simulink model "N4Diag"  (R2024b)
settings: Solver=ode45  StartTime=0.0  StopTime=2  RelTol=1e-3
values from neighbouring files (symbols this model uses):
  T = 10e-3    (= 0.01)    [AnalisisReg.m]    (also in regdiagsep.m = Reg.Ts)
undefined symbols (not defined in the file or in its folder): DiscIntNeverNeededParam, N, RegDiagA_Len2_ext, RegDiagA_Len3_ext, RegDiagA_Len4_ext, RegDiagB_Len2_ext, RegDiagB_Len3_ext, RegDiagB_Len4_ext, RegDiagC_Len2_ext, RegDiagC_Len3_ext, RegDiagC_Len4_ext, RegDiagD_Len2_ext, RegDiagD_Len3_ext, RegDiagD_Len4_ext, RegDiagE_Len2_ext, RegDiagE_Len3_ext, RegDiagE_Len4_ext, RegDiagF_Len2_ext, RegDiagF_Len3_ext, RegDiagF_Len4_ext, RegDiagG_Len2_ext, RegDiagG_Len3_ext, RegDiagG_Len4_ext
libraries: cstblocks x27
settings Model: Creator=Guillem  LastModifiedBy=jroigro
settings SolverCC: AlgebraicLoopSolver=TrustRegion
settings DataIOCC: LimitDataPoints=on  SaveFormat=Array  SignalLoggingSaveFormat=ModelDataLogs  ReturnWorkspaceOutputs=off
settings OptimizationCC: BlockReduction=off  BooleanDataType=off  LifeSpan=inf
settings DebuggingCC: SaveWithParameterizedLinksMsg=none  UnderspecifiedInitializationDetection=Classic  MergeDetectMultiDrivingBlocksExec=none  SignalResolutionControl=TryResolveAllWithWarning  MultiTaskDSMMsg=warning  MultiTaskCondExecSysMsg=none  UnconnectedInputMsg=warning  UnconnectedOutputMsg=warning  UnconnectedLineMsg=warning  SFUnexpectedBacktrackingDiag=warning  SFNoUnconditionalDefaultTransitionDiag=warning  SFExecutionAtInitializationDiag=none  ArithmeticOperatorsInVariantConditions=warning
settings HardwareCC: ProdBitPerPointer=32  ProdBitPerSizeT=32  ProdBitPerPtrDiffT=32  ProdLargestAtomicFloat=None  ProdIntDivRoundTo=Undefined  ProdEndianess=Unspecified  ProdWordSize=32  ProdHWDeviceType=32-bit Generic  TargetUnknown=on
settings ModelReferenceCC: PropagateSignalLabelsOutOfModel=off
settings SFSimCC: SimUseLocalCustomCode=off  CustomCodeUndefinedFunction=UseInterfaceOnly
settings RTWCC: RTWUseLocalCustomCode=off  GPUComputeCapability=3.5
settings CodeAppCC: StateflowObjectComments=on
settings GRTTargetCC: TargetLangStandard=C89/C90 (ANSI)
settings ConfigComp: CovMetricSettings=dw  CovSaveCumulativeToWorkspaceVar=on  CovSaveSingleToWorkspaceVar=on  CovExternalEMLEnable=off

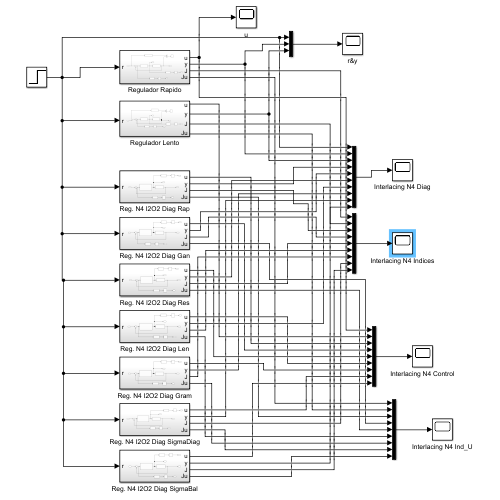
[thumbnail: Simulink's stored preview of the top-level diagram]
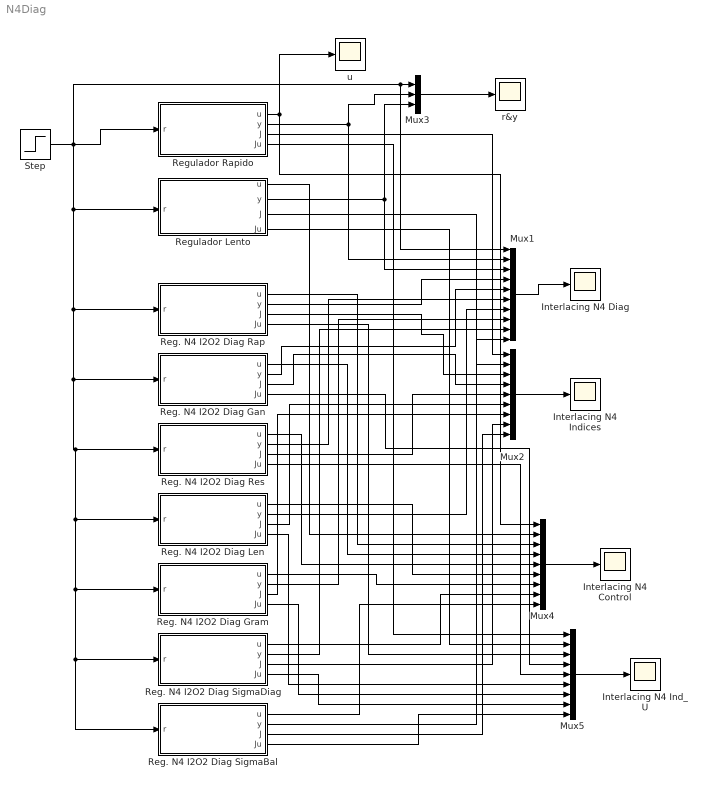
== system N4Diag ==
  Interlacing N4 Control : Scope
  Interlacing N4 Diag : Scope
  Interlacing N4 Ind_U : Scope
  Interlacing N4 Indices : Scope
  Mux1 : Mux  Inputs=10
  Mux2 : Mux  Inputs=9
  Mux3 : Mux  Inputs=3
  Mux4 : Mux  Inputs=9
  Mux5 : Mux  Inputs=9
  Reg. N4 I2O2 Diag Gan : Subsystem
  Reg. N4 I2O2 Diag Gram : Subsystem
  Reg. N4 I2O2 Diag Len : Subsystem
  Reg. N4 I2O2 Diag Rap : Subsystem
  Reg. N4 I2O2 Diag Res : Subsystem
  Reg. N4 I2O2 Diag SigmaBal : Subsystem
  Reg. N4 I2O2 Diag SigmaDiag : Subsystem
  Regulador Lento : Subsystem
  Regulador Rapido : Subsystem
  Step : Step  Time=10  Before=1  After=2  SampleTime=0
  r&y : Scope
  u : Scope
  wires:
  Mux3/1 -> r&y/1
  Regulador Rapido/2(y) -> Mux1/2, Mux3/2
  Regulador Rapido/1(u) -> Mux4/1, u/1
  Mux1/1 -> Interlacing N4 Diag/1
  Regulador Lento/2(y) -> Mux1/3, Mux3/3
  Reg. N4 I2O2 Diag Rap/2(y) -> Mux1/4
  Reg. N4 I2O2 Diag Gan/2(y) -> Mux1/5
  Reg. N4 I2O2 Diag Res/2(y) -> Mux1/6
  Reg. N4 I2O2 Diag Len/2(y) -> Mux1/7
  Mux2/1 -> Interlacing N4 Indices/1
  Regulador Rapido/3(J) -> Mux2/1
  Regulador Lento/3(J) -> Mux2/2
  Reg. N4 I2O2 Diag Rap/3(J) -> Mux2/3
  Reg. N4 I2O2 Diag Gan/3(J) -> Mux2/4
  Reg. N4 I2O2 Diag Res/3(J) -> Mux2/5
  Reg. N4 I2O2 Diag Len/3(J) -> Mux2/6
  Reg. N4 I2O2 Diag Gram/3(J) -> Mux2/7
  Step/1 -> Reg. N4 I2O2 Diag SigmaBal/1(r), Reg. N4 I2O2 Diag SigmaDiag/1(r), Reg. N4 I2O2 Diag Gram/1(r), Reg. N4 I2O2 Diag Len/1(r), Reg. N4 I2O2 Diag Res/1(r), Reg. N4 I2O2 Diag Gan/1(r), Reg. N4 I2O2 Diag Rap/1(r), Regulador Lento/1(r), Mux1/1, Mux3/1, Regulador Rapido/1(r)
  Reg. N4 I2O2 Diag Gram/2(y) -> Mux1/8
  Mux4/1 -> Interlacing N4 Control/1
  Regulador Lento/1(u) -> Mux4/2
  Reg. N4 I2O2 Diag Rap/1(u) -> Mux4/3
  Reg. N4 I2O2 Diag Gan/1(u) -> Mux4/4
  Reg. N4 I2O2 Diag Res/1(u) -> Mux4/5
  Reg. N4 I2O2 Diag Len/1(u) -> Mux4/6
  Reg. N4 I2O2 Diag Gram/1(u) -> Mux4/7
  Reg. N4 I2O2 Diag SigmaDiag/1(u) -> Mux4/8
  Reg. N4 I2O2 Diag SigmaBal/1(u) -> Mux4/9
  Reg. N4 I2O2 Diag SigmaDiag/2(y) -> Mux1/9
  Reg. N4 I2O2 Diag SigmaBal/2(y) -> Mux1/10
  Reg. N4 I2O2 Diag SigmaDiag/3(J) -> Mux2/8
  Reg. N4 I2O2 Diag SigmaBal/3(J) -> Mux2/9
  Mux5/1 -> Interlacing N4 Ind_U/1
  Reg. N4 I2O2 Diag SigmaBal/4(Ju) -> Mux5/9
  Reg. N4 I2O2 Diag SigmaDiag/4(Ju) -> Mux5/8
  Reg. N4 I2O2 Diag Gram/4(Ju) -> Mux5/7
  Reg. N4 I2O2 Diag Len/4(Ju) -> Mux5/6
  Reg. N4 I2O2 Diag Res/4(Ju) -> Mux5/5
  Reg. N4 I2O2 Diag Gan/4(Ju) -> Mux5/4
  Reg. N4 I2O2 Diag Rap/4(Ju) -> Mux5/3
  Regulador Lento/4(Ju) -> Mux5/2
  Regulador Rapido/4(Ju) -> Mux5/1

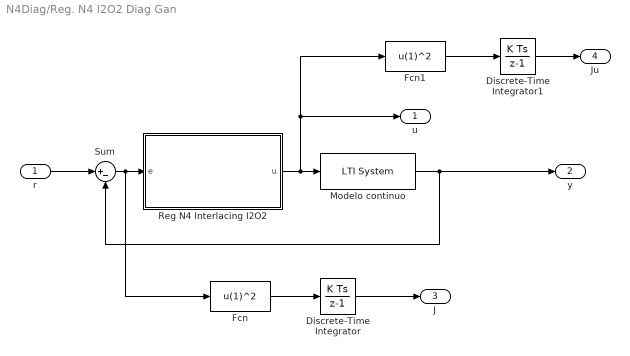
== system N4Diag/Reg. N4 I2O2 Diag Gan ==
  r : Inport
  Discrete-Time Integrator : DiscreteIntegrator  gainval=1/T  SampleTime=T  ICPrevOutput=DiscIntNeverNeededParam  ICPrevScaledInput=DiscIntNeverNeededParam
  Discrete-Time Integrator1 : DiscreteIntegrator  gainval=1/T  SampleTime=T  ICPrevOutput=DiscIntNeverNeededParam  ICPrevScaledInput=DiscIntNeverNeededParam
  Fcn : Fcn  Expr=u(1)^2
  Fcn1 : Fcn  Expr=u(1)^2
  Modelo continuo : cstblocks/LTI System  sys=Planta  IC=[]  PadeOrder=0
  Reg N4 Interlacing I2O2 : Subsystem
  Sum : Sum  Inputs=|+-
  u : Outport
  y : Outport  Port=2
  J : Outport  Port=3
  Ju : Outport  Port=4
  wires:
  r/1 -> Sum/1
  Reg N4 Interlacing I2O2/1(u) -> Fcn1/1, u/1, Modelo continuo/1
  Modelo continuo/1 -> y/1, Sum/2
  Sum/1 -> Fcn/1, Reg N4 Interlacing I2O2/1(e)
  Fcn/1 -> Discrete-Time Integrator/1
  Discrete-Time Integrator/1 -> J/1
  Fcn1/1 -> Discrete-Time Integrator1/1
  Discrete-Time Integrator1/1 -> Ju/1

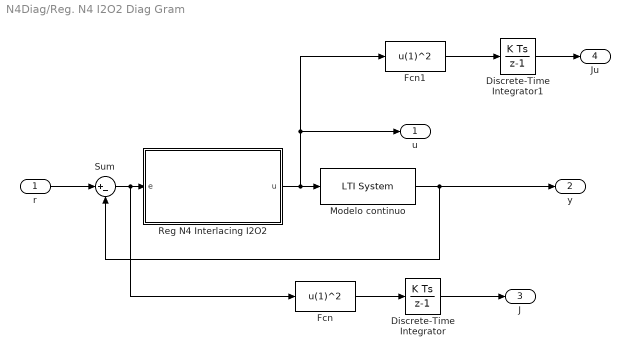
== system N4Diag/Reg. N4 I2O2 Diag Gram ==
  r : Inport
  Discrete-Time Integrator : DiscreteIntegrator  gainval=1/T  SampleTime=T  ICPrevOutput=DiscIntNeverNeededParam  ICPrevScaledInput=DiscIntNeverNeededParam
  Discrete-Time Integrator1 : DiscreteIntegrator  gainval=1/T  SampleTime=T  ICPrevOutput=DiscIntNeverNeededParam  ICPrevScaledInput=DiscIntNeverNeededParam
  Fcn : Fcn  Expr=u(1)^2
  Fcn1 : Fcn  Expr=u(1)^2
  Modelo continuo : cstblocks/LTI System  sys=Planta  IC=[]  PadeOrder=0
  Reg N4 Interlacing I2O2 : Subsystem
  Sum : Sum  Inputs=|+-
  u : Outport
  y : Outport  Port=2
  J : Outport  Port=3
  Ju : Outport  Port=4
  wires:
  Discrete-Time Integrator/1 -> J/1
  Fcn/1 -> Discrete-Time Integrator/1
  Sum/1 -> Reg N4 Interlacing I2O2/1(e), Fcn/1
  Modelo continuo/1 -> Sum/2, y/1
  r/1 -> Sum/1
  Fcn1/1 -> Discrete-Time Integrator1/1
  Reg N4 Interlacing I2O2/1(u) -> Modelo continuo/1, Fcn1/1, u/1
  Discrete-Time Integrator1/1 -> Ju/1

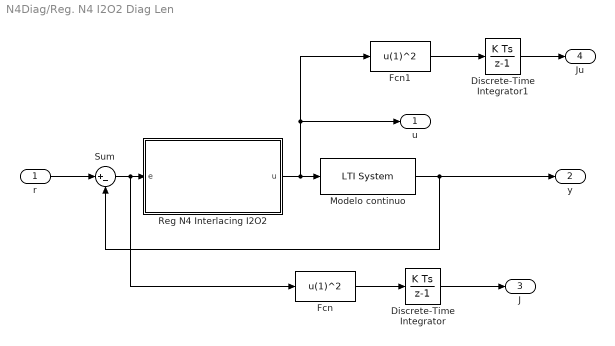
== system N4Diag/Reg. N4 I2O2 Diag Len ==
  r : Inport
  Discrete-Time Integrator : DiscreteIntegrator  gainval=1/T  SampleTime=T  ICPrevOutput=DiscIntNeverNeededParam  ICPrevScaledInput=DiscIntNeverNeededParam
  Discrete-Time Integrator1 : DiscreteIntegrator  gainval=1/T  SampleTime=T  ICPrevOutput=DiscIntNeverNeededParam  ICPrevScaledInput=DiscIntNeverNeededParam
  Fcn : Fcn  Expr=u(1)^2
  Fcn1 : Fcn  Expr=u(1)^2
  Modelo continuo : cstblocks/LTI System  sys=Planta  IC=[]  PadeOrder=0
  Reg N4 Interlacing I2O2 : Subsystem
  Sum : Sum  Inputs=|+-
  u : Outport
  y : Outport  Port=2
  J : Outport  Port=3
  Ju : Outport  Port=4
  wires:
  r/1 -> Sum/1
  Modelo continuo/1 -> y/1, Sum/2
  Sum/1 -> Fcn/1, Reg N4 Interlacing I2O2/1(e)
  Fcn/1 -> Discrete-Time Integrator/1
  Discrete-Time Integrator/1 -> J/1
  Fcn1/1 -> Discrete-Time Integrator1/1
  Reg N4 Interlacing I2O2/1(u) -> Fcn1/1, u/1, Modelo continuo/1
  Discrete-Time Integrator1/1 -> Ju/1

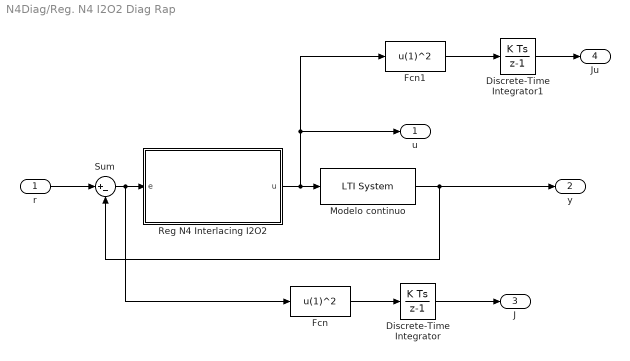
== system N4Diag/Reg. N4 I2O2 Diag Rap ==
  r : Inport
  Discrete-Time Integrator : DiscreteIntegrator  gainval=1/T  SampleTime=T  ICPrevOutput=DiscIntNeverNeededParam  ICPrevScaledInput=DiscIntNeverNeededParam
  Discrete-Time Integrator1 : DiscreteIntegrator  gainval=1/T  SampleTime=T  ICPrevOutput=DiscIntNeverNeededParam  ICPrevScaledInput=DiscIntNeverNeededParam
  Fcn : Fcn  Expr=u(1)^2
  Fcn1 : Fcn  Expr=u(1)^2
  Modelo continuo : cstblocks/LTI System  sys=Planta  IC=[]  PadeOrder=0
  Reg N4 Interlacing I2O2 : Subsystem
  Sum : Sum  Inputs=|+-
  u : Outport
  y : Outport  Port=2
  J : Outport  Port=3
  Ju : Outport  Port=4
  wires:
  Modelo continuo/1 -> Sum/2, y/1
  r/1 -> Sum/1
  Sum/1 -> Fcn/1, Reg N4 Interlacing I2O2/1(e)
  Fcn/1 -> Discrete-Time Integrator/1
  Discrete-Time Integrator/1 -> J/1
  Fcn1/1 -> Discrete-Time Integrator1/1
  Reg N4 Interlacing I2O2/1(u) -> Modelo continuo/1, Fcn1/1, u/1
  Discrete-Time Integrator1/1 -> Ju/1

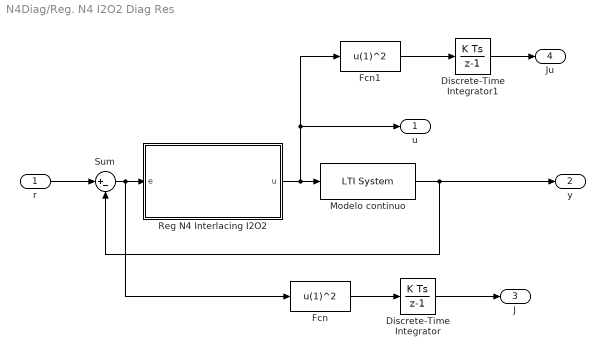
== system N4Diag/Reg. N4 I2O2 Diag Res ==
  r : Inport
  Discrete-Time Integrator : DiscreteIntegrator  gainval=1/T  SampleTime=T  ICPrevOutput=DiscIntNeverNeededParam  ICPrevScaledInput=DiscIntNeverNeededParam
  Discrete-Time Integrator1 : DiscreteIntegrator  gainval=1/T  SampleTime=T  ICPrevOutput=DiscIntNeverNeededParam  ICPrevScaledInput=DiscIntNeverNeededParam
  Fcn : Fcn  Expr=u(1)^2
  Fcn1 : Fcn  Expr=u(1)^2
  Modelo continuo : cstblocks/LTI System  sys=Planta  IC=[]  PadeOrder=0
  Reg N4 Interlacing I2O2 : Subsystem
  Sum : Sum  Inputs=|+-
  u : Outport
  y : Outport  Port=2
  J : Outport  Port=3
  Ju : Outport  Port=4
  wires:
  Modelo continuo/1 -> Sum/2, y/1
  r/1 -> Sum/1
  Sum/1 -> Fcn/1, Reg N4 Interlacing I2O2/1(e)
  Fcn/1 -> Discrete-Time Integrator/1
  Discrete-Time Integrator/1 -> J/1
  Fcn1/1 -> Discrete-Time Integrator1/1
  Reg N4 Interlacing I2O2/1(u) -> Modelo continuo/1, Fcn1/1, u/1
  Discrete-Time Integrator1/1 -> Ju/1

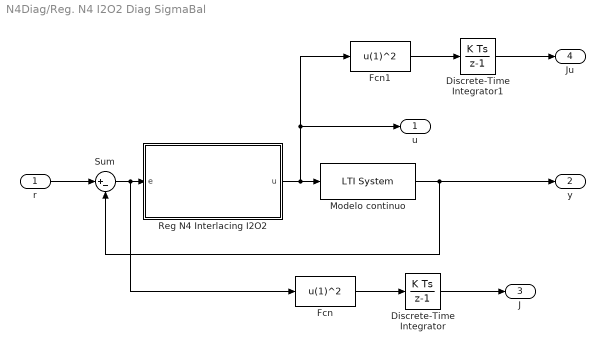
== system N4Diag/Reg. N4 I2O2 Diag SigmaBal ==
  r : Inport
  Discrete-Time Integrator : DiscreteIntegrator  gainval=1/T  SampleTime=T  ICPrevOutput=DiscIntNeverNeededParam  ICPrevScaledInput=DiscIntNeverNeededParam
  Discrete-Time Integrator1 : DiscreteIntegrator  gainval=1/T  SampleTime=T  ICPrevOutput=DiscIntNeverNeededParam  ICPrevScaledInput=DiscIntNeverNeededParam
  Fcn : Fcn  Expr=u(1)^2
  Fcn1 : Fcn  Expr=u(1)^2
  Modelo continuo : cstblocks/LTI System  sys=Planta  IC=[]  PadeOrder=0
  Reg N4 Interlacing I2O2 : Subsystem
  Sum : Sum  Inputs=|+-
  u : Outport
  y : Outport  Port=2
  J : Outport  Port=3
  Ju : Outport  Port=4
  wires:
  r/1 -> Sum/1
  Modelo continuo/1 -> y/1, Sum/2
  Sum/1 -> Fcn/1, Reg N4 Interlacing I2O2/1(e)
  Fcn/1 -> Discrete-Time Integrator/1
  Discrete-Time Integrator/1 -> J/1
  Fcn1/1 -> Discrete-Time Integrator1/1
  Reg N4 Interlacing I2O2/1(u) -> Fcn1/1, u/1, Modelo continuo/1
  Discrete-Time Integrator1/1 -> Ju/1

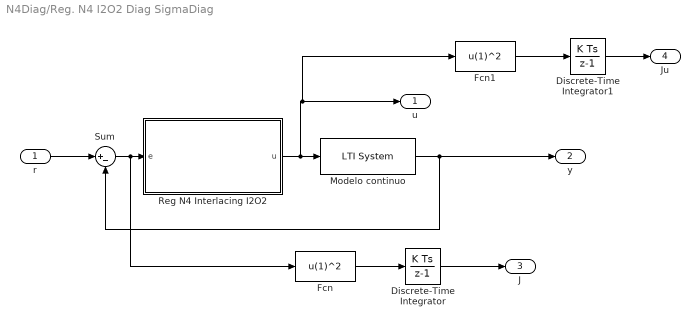
== system N4Diag/Reg. N4 I2O2 Diag SigmaDiag ==
  r : Inport
  Discrete-Time Integrator : DiscreteIntegrator  gainval=1/T  SampleTime=T  ICPrevOutput=DiscIntNeverNeededParam  ICPrevScaledInput=DiscIntNeverNeededParam
  Discrete-Time Integrator1 : DiscreteIntegrator  gainval=1/T  SampleTime=T  ICPrevOutput=DiscIntNeverNeededParam  ICPrevScaledInput=DiscIntNeverNeededParam
  Fcn : Fcn  Expr=u(1)^2
  Fcn1 : Fcn  Expr=u(1)^2
  Modelo continuo : cstblocks/LTI System  sys=Planta  IC=[]  PadeOrder=0
  Reg N4 Interlacing I2O2 : Subsystem
  Sum : Sum  Inputs=|+-
  u : Outport
  y : Outport  Port=2
  J : Outport  Port=3
  Ju : Outport  Port=4
  wires:
  Discrete-Time Integrator/1 -> J/1
  Fcn/1 -> Discrete-Time Integrator/1
  Sum/1 -> Reg N4 Interlacing I2O2/1(e), Fcn/1
  Modelo continuo/1 -> Sum/2, y/1
  r/1 -> Sum/1
  Fcn1/1 -> Discrete-Time Integrator1/1
  Reg N4 Interlacing I2O2/1(u) -> Modelo continuo/1, Fcn1/1, u/1
  Discrete-Time Integrator1/1 -> Ju/1

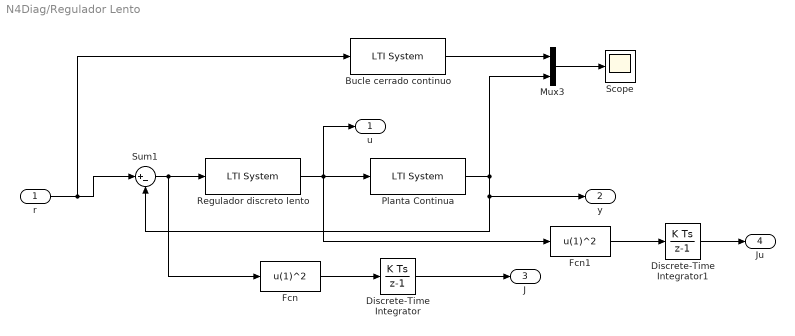
== system N4Diag/Regulador Lento ==
  r : Inport
  Bucle cerrado continuo : cstblocks/LTI System  sys=BC2  IC=[]  PadeOrder=0
  Discrete-Time Integrator : DiscreteIntegrator  gainval=1/T  SampleTime=T  ICPrevOutput=DiscIntNeverNeededParam  ICPrevScaledInput=DiscIntNeverNeededParam
  Discrete-Time Integrator1 : DiscreteIntegrator  gainval=1/T  SampleTime=T  ICPrevOutput=DiscIntNeverNeededParam  ICPrevScaledInput=DiscIntNeverNeededParam
  Fcn : Fcn  Expr=u(1)^2
  Fcn1 : Fcn  Expr=u(1)^2
  Mux3 : Mux  Inputs=2
  Planta Continua : cstblocks/LTI System  sys=Planta  IC=[]  PadeOrder=0
  Regulador discreto lento : cstblocks/LTI System  sys=GrN4  IC=[]  PadeOrder=0
  Scope : Scope
  Sum1 : Sum  Inputs=|+-
  u : Outport
  y : Outport  Port=2
  J : Outport  Port=3
  Ju : Outport  Port=4
  wires:
  r/1 -> Bucle cerrado continuo/1, Sum1/1
  Planta Continua/1 -> Sum1/2, y/1, Mux3/2
  Mux3/1 -> Scope/1
  Bucle cerrado continuo/1 -> Mux3/1
  Sum1/1 -> Fcn/1, Regulador discreto lento/1
  Fcn/1 -> Discrete-Time Integrator/1
  Discrete-Time Integrator/1 -> J/1
  Fcn1/1 -> Discrete-Time Integrator1/1
  Regulador discreto lento/1 -> Fcn1/1, u/1, Planta Continua/1
  Discrete-Time Integrator1/1 -> Ju/1

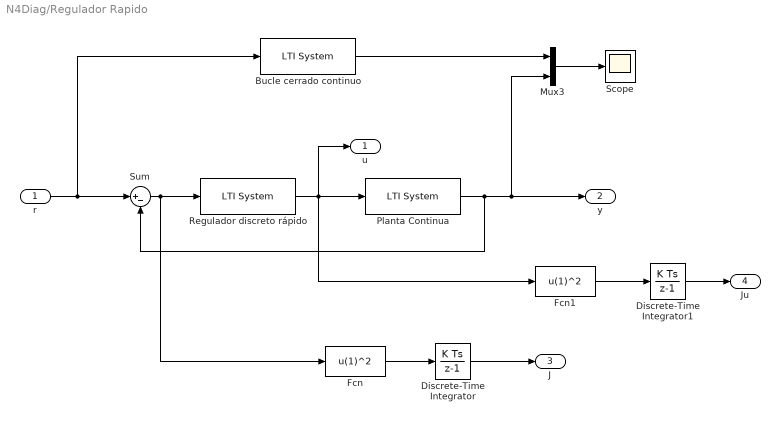
== system N4Diag/Regulador Rapido ==
  r : Inport
  Bucle cerrado continuo : cstblocks/LTI System  sys=BC1  IC=[]  PadeOrder=0
  Discrete-Time Integrator : DiscreteIntegrator  gainval=1/T  SampleTime=T  ICPrevOutput=DiscIntNeverNeededParam  ICPrevScaledInput=DiscIntNeverNeededParam
  Discrete-Time Integrator1 : DiscreteIntegrator  gainval=1/T  SampleTime=T  ICPrevOutput=DiscIntNeverNeededParam  ICPrevScaledInput=DiscIntNeverNeededParam
  Fcn : Fcn  Expr=u(1)^2
  Fcn1 : Fcn  Expr=u(1)^2
  Mux3 : Mux  Inputs=2
  Planta Continua : cstblocks/LTI System  sys=Planta  IC=[]  PadeOrder=0
  Regulador discreto rápido : cstblocks/LTI System  sys=Gr  IC=[]  PadeOrder=0
  Scope : Scope
  Sum : Sum  Inputs=|+-
  u : Outport
  y : Outport  Port=2
  J : Outport  Port=3
  Ju : Outport  Port=4
  wires:
  Bucle cerrado continuo/1 -> Mux3/1
  Mux3/1 -> Scope/1
  Planta Continua/1 -> Mux3/2, y/1, Sum/2
  r/1 -> Sum/1, Bucle cerrado continuo/1
  Discrete-Time Integrator/1 -> J/1
  Sum/1 -> Fcn/1, Regulador discreto rápido/1
  Fcn/1 -> Discrete-Time Integrator/1
  Discrete-Time Integrator1/1 -> Ju/1
  Fcn1/1 -> Discrete-Time Integrator1/1
  Regulador discreto rápido/1 -> Fcn1/1, u/1, Planta Continua/1

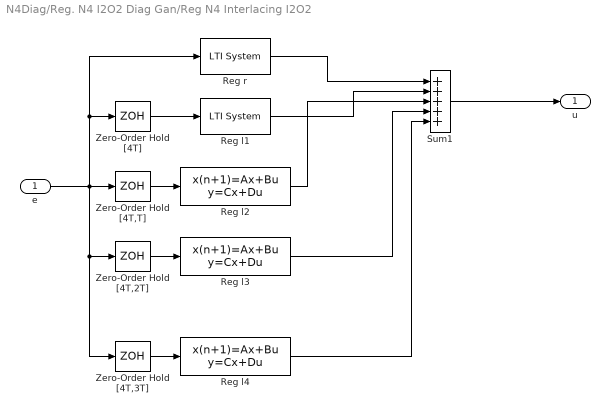
== system N4Diag/Reg. N4 I2O2 Diag Gan/Reg N4 Interlacing I2O2 ==
  e : Inport
  Reg l1 : cstblocks/LTI System  sys=RegDiagB_Len1_ext  IC=[]  PadeOrder=0
  Reg l2 : DiscreteStateSpace  A=RegDiagB_Len2_ext.A  B=RegDiagB_Len2_ext.B  C=RegDiagB_Len2_ext.C  D=RegDiagB_Len2_ext.D  SampleTime=[N*T,T]
  Reg l3 : DiscreteStateSpace  A=RegDiagB_Len3_ext.A  B=RegDiagB_Len3_ext.B  C=RegDiagB_Len3_ext.C  D=RegDiagB_Len3_ext.D  SampleTime=[N*T,2*T]
  Reg l4 : DiscreteStateSpace  A=RegDiagB_Len4_ext.A  B=RegDiagB_Len4_ext.B  C=RegDiagB_Len4_ext.C  D=RegDiagB_Len4_ext.D  SampleTime=[N*T,3*T]
  Reg r : cstblocks/LTI System  sys=RegDiagB_Rap  IC=[]  PadeOrder=0
  Sum1 : Sum  Inputs=+++++
  Zero-Order Hold [4T,2T] : ZeroOrderHold  SampleTime=[N*T,2*T]
  Zero-Order Hold [4T,3T] : ZeroOrderHold  SampleTime=[N*T,3*T]
  Zero-Order Hold [4T,T] : ZeroOrderHold  SampleTime=[N*T,T]
  Zero-Order Hold [4T] : ZeroOrderHold  SampleTime=[N*T]
  u : Outport
  wires:
  Reg l4/1 -> Sum1/5
  e/1 -> Reg r/1, Zero-Order Hold [4T]/1, Zero-Order Hold [4T,T]/1, Zero-Order Hold [4T,2T]/1, Zero-Order Hold [4T,3T]/1
  Zero-Order Hold [4T,3T]/1 -> Reg l4/1
  Reg l3/1 -> Sum1/4
  Zero-Order Hold [4T,2T]/1 -> Reg l3/1
  Zero-Order Hold [4T]/1 -> Reg l1/1
  Zero-Order Hold [4T,T]/1 -> Reg l2/1
  Sum1/1 -> u/1
  Reg l1/1 -> Sum1/2
  Reg r/1 -> Sum1/1
  Reg l2/1 -> Sum1/3

== system N4Diag/Reg. N4 I2O2 Diag Gram/Reg N4 Interlacing I2O2 ==
  e : Inport
  Reg l1 : cstblocks/LTI System  sys=RegDiagE_Len1_ext  IC=[]  PadeOrder=0
  Reg l2 : DiscreteStateSpace  A=RegDiagE_Len2_ext.A  B=RegDiagE_Len2_ext.B  C=RegDiagE_Len2_ext.C  D=RegDiagE_Len2_ext.D  SampleTime=[N*T,T]
  Reg l3 : DiscreteStateSpace  A=RegDiagE_Len3_ext.A  B=RegDiagE_Len3_ext.B  C=RegDiagE_Len3_ext.C  D=RegDiagE_Len3_ext.D  SampleTime=[N*T,2*T]
  Reg l4 : DiscreteStateSpace  A=RegDiagE_Len4_ext.A  B=RegDiagE_Len4_ext.B  C=RegDiagE_Len4_ext.C  D=RegDiagE_Len4_ext.D  SampleTime=[N*T,3*T]
  Reg r : cstblocks/LTI System  sys=RegDiagE_Rap  IC=[]  PadeOrder=0
  Sum1 : Sum  Inputs=+++++
  Zero-Order Hold [4T,2T] : ZeroOrderHold  SampleTime=[N*T,2*T]
  Zero-Order Hold [4T,3T] : ZeroOrderHold  SampleTime=[N*T,3*T]
  Zero-Order Hold [4T,T] : ZeroOrderHold  SampleTime=[N*T,T]
  Zero-Order Hold [4T] : ZeroOrderHold  SampleTime=[N*T]
  u : Outport
  wires:
  Reg l2/1 -> Sum1/3
  Reg r/1 -> Sum1/1
  Reg l1/1 -> Sum1/2
  Sum1/1 -> u/1
  Zero-Order Hold [4T,T]/1 -> Reg l2/1
  Zero-Order Hold [4T]/1 -> Reg l1/1
  Zero-Order Hold [4T,2T]/1 -> Reg l3/1
  Reg l3/1 -> Sum1/4
  Zero-Order Hold [4T,3T]/1 -> Reg l4/1
  e/1 -> Zero-Order Hold [4T,T]/1, Zero-Order Hold [4T,3T]/1, Zero-Order Hold [4T,2T]/1, Zero-Order Hold [4T]/1, Reg r/1
  Reg l4/1 -> Sum1/5

== system N4Diag/Reg. N4 I2O2 Diag Len/Reg N4 Interlacing I2O2 ==
  e : Inport
  Reg l1 : cstblocks/LTI System  sys=RegDiagD_Len1_ext  IC=[]  PadeOrder=0
  Reg l2 : DiscreteStateSpace  A=RegDiagD_Len2_ext.A  B=RegDiagD_Len2_ext.B  C=RegDiagD_Len2_ext.C  D=RegDiagD_Len2_ext.D  SampleTime=[N*T,T]
  Reg l3 : DiscreteStateSpace  A=RegDiagD_Len3_ext.A  B=RegDiagD_Len3_ext.B  C=RegDiagD_Len3_ext.C  D=RegDiagD_Len3_ext.D  SampleTime=[N*T,2*T]
  Reg l4 : DiscreteStateSpace  A=RegDiagD_Len4_ext.A  B=RegDiagD_Len4_ext.B  C=RegDiagD_Len4_ext.C  D=RegDiagD_Len4_ext.D  SampleTime=[N*T,3*T]
  Reg r : cstblocks/LTI System  sys=RegDiagD_Rap  IC=[]  PadeOrder=0
  Sum1 : Sum  Inputs=+++++
  Zero-Order Hold [4T,2T] : ZeroOrderHold  SampleTime=[N*T,2*T]
  Zero-Order Hold [4T,3T] : ZeroOrderHold  SampleTime=[N*T,3*T]
  Zero-Order Hold [4T,T] : ZeroOrderHold  SampleTime=[N*T,T]
  Zero-Order Hold [4T] : ZeroOrderHold  SampleTime=[N*T]
  u : Outport
  wires:
  Reg l4/1 -> Sum1/5
  e/1 -> Reg r/1, Zero-Order Hold [4T]/1, Zero-Order Hold [4T,T]/1, Zero-Order Hold [4T,2T]/1, Zero-Order Hold [4T,3T]/1
  Zero-Order Hold [4T,3T]/1 -> Reg l4/1
  Reg l3/1 -> Sum1/4
  Zero-Order Hold [4T,2T]/1 -> Reg l3/1
  Zero-Order Hold [4T]/1 -> Reg l1/1
  Zero-Order Hold [4T,T]/1 -> Reg l2/1
  Sum1/1 -> u/1
  Reg l1/1 -> Sum1/2
  Reg r/1 -> Sum1/1
  Reg l2/1 -> Sum1/3

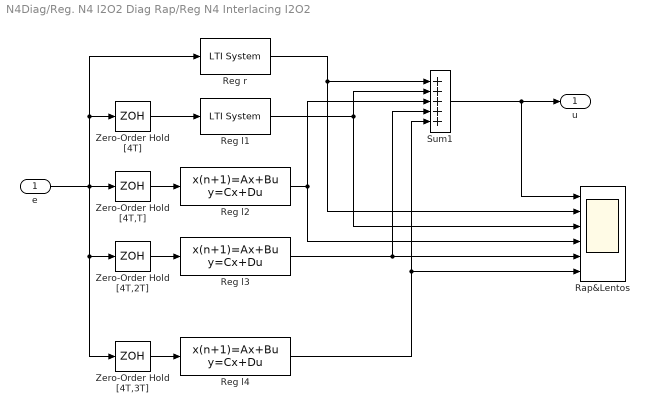
== system N4Diag/Reg. N4 I2O2 Diag Rap/Reg N4 Interlacing I2O2 ==
  e : Inport
  Rap&Lentos : Scope  NumInputPorts=6
  Reg l1 : cstblocks/LTI System  sys=RegDiagA_Len1_ext  IC=[]  PadeOrder=0
  Reg l2 : DiscreteStateSpace  A=RegDiagA_Len2_ext.A  B=RegDiagA_Len2_ext.B  C=RegDiagA_Len2_ext.C  D=RegDiagA_Len2_ext.D  SampleTime=[N*T,T]
  Reg l3 : DiscreteStateSpace  A=RegDiagA_Len3_ext.A  B=RegDiagA_Len3_ext.B  C=RegDiagA_Len3_ext.C  D=RegDiagA_Len3_ext.D  SampleTime=[N*T,2*T]
  Reg l4 : DiscreteStateSpace  A=RegDiagA_Len4_ext.A  B=RegDiagA_Len4_ext.B  C=RegDiagA_Len4_ext.C  D=RegDiagA_Len4_ext.D  SampleTime=[N*T,3*T]
  Reg r : cstblocks/LTI System  sys=RegDiagA_Rap  IC=[]  PadeOrder=0
  Sum1 : Sum  Inputs=+++++
  Zero-Order Hold [4T,2T] : ZeroOrderHold  SampleTime=[N*T,2*T]
  Zero-Order Hold [4T,3T] : ZeroOrderHold  SampleTime=[N*T,3*T]
  Zero-Order Hold [4T,T] : ZeroOrderHold  SampleTime=[N*T,T]
  Zero-Order Hold [4T] : ZeroOrderHold  SampleTime=[N*T]
  u : Outport
  wires:
  Reg l2/1 -> Rap&Lentos/4, Sum1/3
  Reg r/1 -> Rap&Lentos/2, Sum1/1
  Reg l1/1 -> Rap&Lentos/3, Sum1/2
  Sum1/1 -> u/1, Rap&Lentos/1
  Zero-Order Hold [4T,T]/1 -> Reg l2/1
  Zero-Order Hold [4T]/1 -> Reg l1/1
  Zero-Order Hold [4T,2T]/1 -> Reg l3/1
  Reg l3/1 -> Rap&Lentos/5, Sum1/4
  Zero-Order Hold [4T,3T]/1 -> Reg l4/1
  e/1 -> Zero-Order Hold [4T,3T]/1, Zero-Order Hold [4T,2T]/1, Zero-Order Hold [4T,T]/1, Zero-Order Hold [4T]/1, Reg r/1
  Reg l4/1 -> Rap&Lentos/6, Sum1/5

== system N4Diag/Reg. N4 I2O2 Diag Res/Reg N4 Interlacing I2O2 ==
  e : Inport
  Reg l1 : cstblocks/LTI System  sys=RegDiagC_Len1_ext  IC=[]  PadeOrder=0
  Reg l2 : DiscreteStateSpace  A=RegDiagC_Len2_ext.A  B=RegDiagC_Len2_ext.B  C=RegDiagC_Len2_ext.C  D=RegDiagC_Len2_ext.D  SampleTime=[N*T,T]
  Reg l3 : DiscreteStateSpace  A=RegDiagC_Len3_ext.A  B=RegDiagC_Len3_ext.B  C=RegDiagC_Len3_ext.C  D=RegDiagC_Len3_ext.D  SampleTime=[N*T,2*T]
  Reg l4 : DiscreteStateSpace  A=RegDiagC_Len4_ext.A  B=RegDiagC_Len4_ext.B  C=RegDiagC_Len4_ext.C  D=RegDiagC_Len4_ext.D  SampleTime=[N*T,3*T]
  Reg r : cstblocks/LTI System  sys=RegDiagC_Rap  IC=[]  PadeOrder=0
  Sum1 : Sum  Inputs=+++++
  Zero-Order Hold [4T,2T] : ZeroOrderHold  SampleTime=[N*T,2*T]
  Zero-Order Hold [4T,3T] : ZeroOrderHold  SampleTime=[N*T,3*T]
  Zero-Order Hold [4T,T] : ZeroOrderHold  SampleTime=[N*T,T]
  Zero-Order Hold [4T] : ZeroOrderHold  SampleTime=[N*T]
  u : Outport
  wires:
  Reg l2/1 -> Sum1/3
  Reg r/1 -> Sum1/1
  Reg l1/1 -> Sum1/2
  Sum1/1 -> u/1
  Zero-Order Hold [4T,T]/1 -> Reg l2/1
  Zero-Order Hold [4T]/1 -> Reg l1/1
  Zero-Order Hold [4T,2T]/1 -> Reg l3/1
  Reg l3/1 -> Sum1/4
  Zero-Order Hold [4T,3T]/1 -> Reg l4/1
  e/1 -> Zero-Order Hold [4T,3T]/1, Zero-Order Hold [4T,2T]/1, Zero-Order Hold [4T,T]/1, Zero-Order Hold [4T]/1, Reg r/1
  Reg l4/1 -> Sum1/5

== system N4Diag/Reg. N4 I2O2 Diag SigmaBal/Reg N4 Interlacing I2O2 ==
  e : Inport
  Reg l1 : cstblocks/LTI System  sys=RegDiagF_Len1_ext  IC=[]  PadeOrder=0
  Reg l2 : DiscreteStateSpace  A=RegDiagF_Len2_ext.A  B=RegDiagF_Len2_ext.B  C=RegDiagF_Len2_ext.C  D=RegDiagF_Len2_ext.D  SampleTime=[N*T,T]
  Reg l3 : DiscreteStateSpace  A=RegDiagF_Len3_ext.A  B=RegDiagF_Len3_ext.B  C=RegDiagF_Len3_ext.C  D=RegDiagF_Len3_ext.D  SampleTime=[N*T,2*T]
  Reg l4 : DiscreteStateSpace  A=RegDiagF_Len4_ext.A  B=RegDiagF_Len4_ext.B  C=RegDiagF_Len4_ext.C  D=RegDiagF_Len4_ext.D  SampleTime=[N*T,3*T]
  Reg r : cstblocks/LTI System  sys=RegDiagF_Rap  IC=[]  PadeOrder=0
  Sum1 : Sum  Inputs=+++++
  Zero-Order Hold [4T,2T] : ZeroOrderHold  SampleTime=[N*T,2*T]
  Zero-Order Hold [4T,3T] : ZeroOrderHold  SampleTime=[N*T,3*T]
  Zero-Order Hold [4T,T] : ZeroOrderHold  SampleTime=[N*T,T]
  Zero-Order Hold [4T] : ZeroOrderHold  SampleTime=[N*T]
  u : Outport
  wires:
  Reg l4/1 -> Sum1/5
  e/1 -> Reg r/1, Zero-Order Hold [4T]/1, Zero-Order Hold [4T,2T]/1, Zero-Order Hold [4T,3T]/1, Zero-Order Hold [4T,T]/1
  Zero-Order Hold [4T,3T]/1 -> Reg l4/1
  Reg l3/1 -> Sum1/4
  Zero-Order Hold [4T,2T]/1 -> Reg l3/1
  Zero-Order Hold [4T]/1 -> Reg l1/1
  Zero-Order Hold [4T,T]/1 -> Reg l2/1
  Sum1/1 -> u/1
  Reg l1/1 -> Sum1/2
  Reg r/1 -> Sum1/1
  Reg l2/1 -> Sum1/3

== system N4Diag/Reg. N4 I2O2 Diag SigmaDiag/Reg N4 Interlacing I2O2 ==
  e : Inport
  Reg l1 : cstblocks/LTI System  sys=RegDiagG_Len1_ext  IC=[]  PadeOrder=0
  Reg l2 : DiscreteStateSpace  A=RegDiagG_Len2_ext.A  B=RegDiagG_Len2_ext.B  C=RegDiagG_Len2_ext.C  D=RegDiagG_Len2_ext.D  SampleTime=[N*T,T]
  Reg l3 : DiscreteStateSpace  A=RegDiagG_Len3_ext.A  B=RegDiagG_Len3_ext.B  C=RegDiagG_Len3_ext.C  D=RegDiagG_Len3_ext.D  SampleTime=[N*T,2*T]
  Reg l4 : DiscreteStateSpace  A=RegDiagG_Len4_ext.A  B=RegDiagG_Len4_ext.B  C=RegDiagG_Len4_ext.C  D=RegDiagG_Len4_ext.D  SampleTime=[N*T,3*T]
  Reg r : cstblocks/LTI System  sys=RegDiagG_Rap  IC=[]  PadeOrder=0
  Sum1 : Sum  Inputs=+++++
  Zero-Order Hold [4T,2T] : ZeroOrderHold  SampleTime=[N*T,2*T]
  Zero-Order Hold [4T,3T] : ZeroOrderHold  SampleTime=[N*T,3*T]
  Zero-Order Hold [4T,T] : ZeroOrderHold  SampleTime=[N*T,T]
  Zero-Order Hold [4T] : ZeroOrderHold  SampleTime=[N*T]
  u : Outport
  wires:
  Reg l2/1 -> Sum1/3
  Reg r/1 -> Sum1/1
  Reg l1/1 -> Sum1/2
  Sum1/1 -> u/1
  Zero-Order Hold [4T,T]/1 -> Reg l2/1
  Zero-Order Hold [4T]/1 -> Reg l1/1
  Zero-Order Hold [4T,2T]/1 -> Reg l3/1
  Reg l3/1 -> Sum1/4
  Zero-Order Hold [4T,3T]/1 -> Reg l4/1
  e/1 -> Zero-Order Hold [4T,T]/1, Zero-Order Hold [4T,3T]/1, Zero-Order Hold [4T,2T]/1, Zero-Order Hold [4T]/1, Reg r/1
  Reg l4/1 -> Sum1/5
